simulink model "drive_plant_ideal"  (R2026b)
settings: Solver=VariableStepAuto
undefined symbols (not defined in the file or in its folder): P
libraries: fl_lib x28, nesl_utility x8, ee_lib x1
settings Model: Creator=aomar  LastModifiedBy=aomar

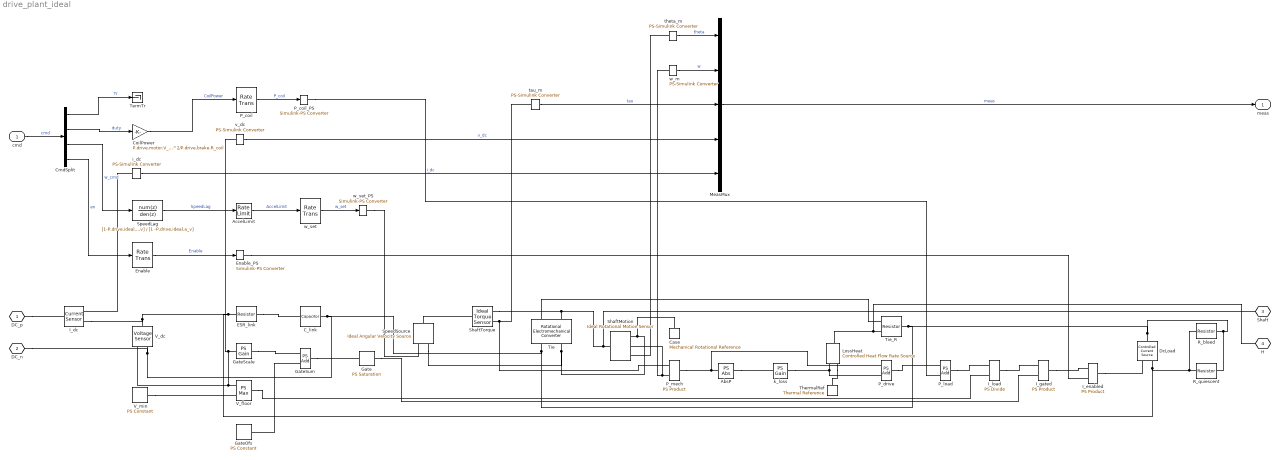
== system drive_plant_ideal ==
  cmd : Inport  OutDataTypeStr=double  SampleTime=P.drive.Ts_esc
  AbsP : fl_lib/Physical Signals/Nonlinear Operators/PS Abs  ZeroCross=true
  AccelLimit : RateLimiter  RisingSlewLimit=P.drive.ideal.a_max  FallingSlewLimit=-P.drive.ideal.a_max  SampleTimeMode=inherited
  C_link : fl_lib/Electrical/Electrical Elements/Capacitor  c=P.drive.esc.C_link F  r=1e-6 Ohm  g=0 1/Ohm  i_specify=off  i_priority=None  i=0 A  i_nominal_specify=off  i_nominal_value=1  i_nominal_unit=A  v_specify=off  v_priority=None  v=0 V  v_nominal_specify=off  v_nominal_value=1  v_nominal_unit=V  vc_specify=on  vc_priority=High  vc=P.drive.esc.vc0 V  vc_nominal_specify=off  vc_nominal_value=1  vc_nominal_unit=V
  Case : fl_lib/Mechanical/Rotational Elements/Mechanical Rotational Reference
  CmdSplit : Demux
  CoilPower : Gain  Gain=P.drive.motor.V_nom^2/P.drive.brake.R_coil
  DcLoad : fl_lib/Electrical/Electrical Sources/Controlled Current Source
  ESR_link : fl_lib/Electrical/Electrical Elements/Resistor  R=P.drive.esc.ESR_link Ohm  i_specify=off  i_priority=None  i=0 A  i_nominal_specify=off  i_nominal_value=1  i_nominal_unit=A  v_specify=off  v_priority=None  v=0 V  v_nominal_specify=off  v_nominal_value=1  v_nominal_unit=V
  Enable : RateTransition  OutPortSampleTimeOpt=Inherit
  Enable_PS : nesl_utility/Simulink-PS Converter  PhysicalDomain=network_engine_domain  SubClassName=ps_input  LeftPortType=input  RightPortType=output  PseudoPeriodic=off  Frequencies=[]  NoiseDistribution=none  NoiseParameters=[]  Unit=1  AffineConversion=off  FilteringAndDerivatives=zero  SimscapeFilterOrder=1  InputFilterTimeConstant=0.001  UdotUserProvided=0
  Gate : fl_lib/Physical Signals/Nonlinear Operators/PS Saturation  upper_limit=1  lower_limit=0  ZeroCross=true
  GateOfs : fl_lib/Physical Signals/Sources/PS Constant  constant=-(P.drive.ideal.V_min - P.drive.ideal.V_gate)/P.drive.ideal.V_gate
  GateScale : fl_lib/Physical Signals/Functions/PS Gain  gain=1/P.drive.ideal.V_gate 1/V
  GateSum : fl_lib/Physical Signals/Functions/PS Add
  I_dc : fl_lib/Electrical/Electrical Sensors/Current Sensor
  I_enabled : fl_lib/Physical Signals/Functions/PS Product
  I_gated : fl_lib/Physical Signals/Functions/PS Product
  I_load : fl_lib/Physical Signals/Functions/PS Divide
  LossHeat : fl_lib/Thermal/Thermal Sources/Controlled Heat Flow Rate Source
  MeasMux : Mux  Inputs=5
  P_coil : RateTransition  OutPortSampleTimeOpt=Inherit
  P_coil_PS : nesl_utility/Simulink-PS Converter  PhysicalDomain=network_engine_domain  SubClassName=ps_input  LeftPortType=input  RightPortType=output  PseudoPeriodic=off  Frequencies=[]  NoiseDistribution=none  NoiseParameters=[]  Unit=W  AffineConversion=off  FilteringAndDerivatives=zero  SimscapeFilterOrder=1  InputFilterTimeConstant=0.001  UdotUserProvided=0
  P_drive : fl_lib/Physical Signals/Functions/PS Add
  P_load : fl_lib/Physical Signals/Functions/PS Add
  P_mech : fl_lib/Physical Signals/Functions/PS Product
  R_bleed : fl_lib/Electrical/Electrical Elements/Resistor  R=P.drive.esc.R_bleed Ohm  i_specify=off  i_priority=None  i=0 A  i_nominal_specify=off  i_nominal_value=1  i_nominal_unit=A  v_specify=off  v_priority=None  v=0 V  v_nominal_specify=off  v_nominal_value=1  v_nominal_unit=V
  R_quiescent : fl_lib/Electrical/Electrical Elements/Resistor  R=P.drive.esc.R_q Ohm  i_specify=off  i_priority=None  i=0 A  i_nominal_specify=off  i_nominal_value=1  i_nominal_unit=A  v_specify=off  v_priority=None  v=0 V  v_nominal_specify=off  v_nominal_value=1  v_nominal_unit=V
  ShaftMotion : fl_lib/Mechanical/Mechanical Sensors/Ideal Rotational Motion Sensor  reference=foundation.enum.MeasurementReference.difference  acceleration_port=false  velocity_port=true  position_port=true  wrap_angle=false  offset=0 rad
  ShaftTorque : fl_lib/Mechanical/Mechanical Sensors/Ideal Torque Sensor
  SpeedLag : DiscreteTransferFcn  Numerator=[1-P.drive.ideal.a_v]  Denominator=[1 -P.drive.ideal.a_v]  SampleTime=P.drive.Ts_esc
  SpeedSource : fl_lib/Mechanical/Mechanical Sources/Ideal Angular Velocity Source
  TermTr : Terminator
  ThermalRef : fl_lib/Thermal/Thermal Elements/Thermal Reference
  Tie : fl_lib/Electrical/Electrical Elements/Rotational Electromechanical Converter  K=P.drive.tie.K V*s/rad  i_specify=off  i_priority=None  i=0 A  i_nominal_specify=off  i_nominal_value=1  i_nominal_unit=A  v_specify=off  v_priority=None  v=0 V  v_nominal_specify=off  v_nominal_value=1  v_nominal_unit=V  t_specify=off  t_priority=None  t=0 N*m  t_nominal_specify=off  t_nominal_value=1  t_nominal_unit=N*m  w_specify=off  w_priority=None  w=0 rad/s  w_nominal_specify=off  w_nominal_value=1  w_nominal_unit=rad/s
  Tie_R : ee_lib/Passive/Resistor  R=P.drive.tie.R Ohm  enable_R_tol=ee.enum.toleranceApplication.none  R_tol=5  tol_distribution=ee.enum.toleranceDistribution.uniform  nSigma=4  enable_operating_limits=ee.enum.enable.no  operating_limit_action=ee.enum.passive.reportOpLim.warn  power_rating=1 W  max_working_voltage=100 V  noise_mode=ee.enum.sources.noise.Disabled  Tdevice=25 degC  sample_time=1e-3 s  repeatability=ee.enum.ic.repeatability.notRepeatable  user_seed=0  auto_seed=3499211588  power_derating_T1=70 degC  power_derating_T2=155 degC  operating_temperature_range_vec=[-50, 150] degC  alpha=3.93e-3 1/K  Tmeas=25 degC  thermal_mass=P.drive.thermal.C_w J/K  temperature_specify=on  temperature_priority=High  temperature=P.drive.thermal.T_amb0 K  temperature_nominal_specify=off  temperature_nominal_value=1  temperature_nominal_unit=K
  V_dc : fl_lib/Electrical/Electrical Sensors/Voltage Sensor
  V_floor : fl_lib/Physical Signals/Nonlinear Operators/PS Max  ZeroCross=true
  V_min : fl_lib/Physical Signals/Sources/PS Constant  constant=P.drive.ideal.V_min V
  i_dc : nesl_utility/PS-Simulink Converter  PhysicalDomain=network_engine_domain  SubClassName=ps_output  LeftPortType=input  RightPortType=output  PseudoPeriodic=off  Frequencies=[]  VectorFormat=inherit  Unit=A  AffineConversion=off
  k_loss : fl_lib/Physical Signals/Functions/PS Gain  gain=P.drive.ideal.k_loss
  tau_m : nesl_utility/PS-Simulink Converter  PhysicalDomain=network_engine_domain  SubClassName=ps_output  LeftPortType=input  RightPortType=output  PseudoPeriodic=off  Frequencies=[]  VectorFormat=inherit  Unit=N*m  AffineConversion=off
  theta_m : nesl_utility/PS-Simulink Converter  PhysicalDomain=network_engine_domain  SubClassName=ps_output  LeftPortType=input  RightPortType=output  PseudoPeriodic=off  Frequencies=[]  VectorFormat=inherit  Unit=rad  AffineConversion=off
  v_dc : nesl_utility/PS-Simulink Converter  PhysicalDomain=network_engine_domain  SubClassName=ps_output  LeftPortType=input  RightPortType=output  PseudoPeriodic=off  Frequencies=[]  VectorFormat=inherit  Unit=V  AffineConversion=off
  w_m : nesl_utility/PS-Simulink Converter  PhysicalDomain=network_engine_domain  SubClassName=ps_output  LeftPortType=input  RightPortType=output  PseudoPeriodic=off  Frequencies=[]  VectorFormat=inherit  Unit=rad/s  AffineConversion=off
  w_set : RateTransition  OutPortSampleTimeOpt=Inherit
  w_set_PS : nesl_utility/Simulink-PS Converter  PhysicalDomain=network_engine_domain  SubClassName=ps_input  LeftPortType=input  RightPortType=output  PseudoPeriodic=off  Frequencies=[]  NoiseDistribution=none  NoiseParameters=[]  Unit=rad/s  AffineConversion=off  FilteringAndDerivatives=zero  SimscapeFilterOrder=1  InputFilterTimeConstant=0.001  UdotUserProvided=0
  DC_p : PMIOPort  Side=Left  ConnectionType=Connection: foundation.electrical.electrical
  DC_n : PMIOPort  Port=2  Side=Left  ConnectionType=Connection: foundation.electrical.electrical
  Shaft : PMIOPort  Port=3  Side=Right  ConnectionType=Connection: foundation.mechanical.rotational.rotational
  H : PMIOPort  Port=4  Side=Right  ConnectionType=Connection: foundation.thermal.thermal
  meas : Outport  OutDataTypeStr=double
  wires:
  cmd/1 -> CmdSplit/1  "cmd"
  CmdSplit/1 -> TermTr/1  "Tr"
  CmdSplit/2 -> CoilPower/1  "duty"
  CmdSplit/3 -> SpeedLag/1  "w_cmd"
  CmdSplit/4 -> Enable/1  "en"
  i_dc/1 -> MeasMux/5  "i_dc"
  CoilPower/1 -> P_coil/1  "CoilPower"
  Enable/1 -> Enable_PS/1  "Enable"
  SpeedLag/1 -> AccelLimit/1  "SpeedLag"
  v_dc/1 -> MeasMux/4  "v_dc"
  AccelLimit/1 -> w_set/1  "AccelLimit"
  P_coil/1 -> P_coil_PS/1  "P_coil"
  w_set/1 -> w_set_PS/1  "w_set"
  tau_m/1 -> MeasMux/3  "tau"
  theta_m/1 -> MeasMux/1  "theta"
  w_m/1 -> MeasMux/2  "w"
  MeasMux/1 -> meas/1  "meas"
  connections:
  AbsP/LConn1 -- P_mech/RConn1 -- P_drive/LConn1
  AbsP/RConn1 -- k_loss/LConn1
  ESR_link/RConn1 -- C_link/LConn1
  V_dc/RConn2 -- DC_n/RConn1 -- C_link/RConn1 -- Tie/RConn1 -- Tie_R/RConn1 -- DcLoad/LConn1 -- R_bleed/RConn1 -- R_quiescent/RConn1
  Tie/RConn2 -- SpeedSource/RConn2 -- ShaftMotion/RConn1 -- Case/LConn1
  DC_p/RConn1 -- I_dc/LConn1
  I_enabled/RConn1 -- DcLoad/RConn1
  Enable_PS/RConn1 -- I_enabled/LConn2
  GateSum/RConn1 -- Gate/LConn1
  Gate/RConn1 -- I_gated/LConn2
  GateSum/LConn2 -- GateOfs/RConn1
  GateScale/RConn1 -- GateSum/LConn1
  Tie_R/LConn2 -- LossHeat/LConn1 -- H/RConn1
  i_dc/LConn1 -- I_dc/RConn1
  I_gated/RConn1 -- I_enabled/LConn1
  I_load/RConn1 -- I_gated/LConn1
  P_load/RConn1 -- I_load/LConn1
  V_floor/RConn1 -- I_load/LConn2
  LossHeat/RConn1 -- k_loss/RConn1 -- P_drive/LConn2
  LossHeat/RConn2 -- ThermalRef/LConn1
  P_coil_PS/RConn1 -- P_load/LConn2
  P_drive/RConn1 -- P_load/LConn1
  ShaftTorque/RConn2 -- tau_m/LConn1 -- P_mech/LConn1
  P_mech/LConn2 -- w_m/LConn1 -- ShaftMotion/RConn2
  Tie/LConn2 -- ShaftTorque/RConn1 -- ShaftMotion/LConn1 -- Shaft/RConn1
  theta_m/LConn1 -- ShaftMotion/RConn3
  SpeedSource/LConn1 -- ShaftTorque/LConn1
  w_set_PS/RConn1 -- SpeedSource/RConn1
  Tie/LConn1 -- Tie_R/LConn1
  V_min/RConn1 -- V_floor/LConn2
  V_dc/LConn1 -- I_dc/RConn2 -- ESR_link/LConn1 -- DcLoad/RConn2 -- R_quiescent/LConn1 -- R_bleed/LConn1
  GateScale/LConn1 -- v_dc/LConn1 -- V_floor/LConn1 -- V_dc/RConn1
